simulink subsystem "StudentTemplate_MTMTAD006_M1(draft)"  (R2025a)
settings: Solver=VariableStepAuto  StartTime=0.0  StopTime=10.0  RelTol=1e-3
libraries: simulink x6, eeGeneralControl x3, slpidlib x1, cstblocks x1, dspstat3 x1
settings Model: Creator=JesseJabezArendse  LastModifiedBy=MTMTAD006

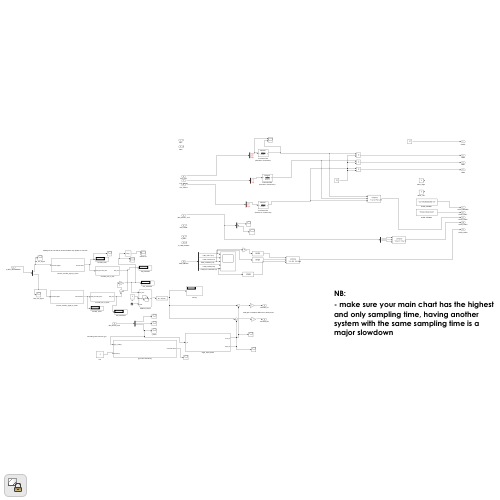
[thumbnail: Simulink's stored preview of the top-level diagram]
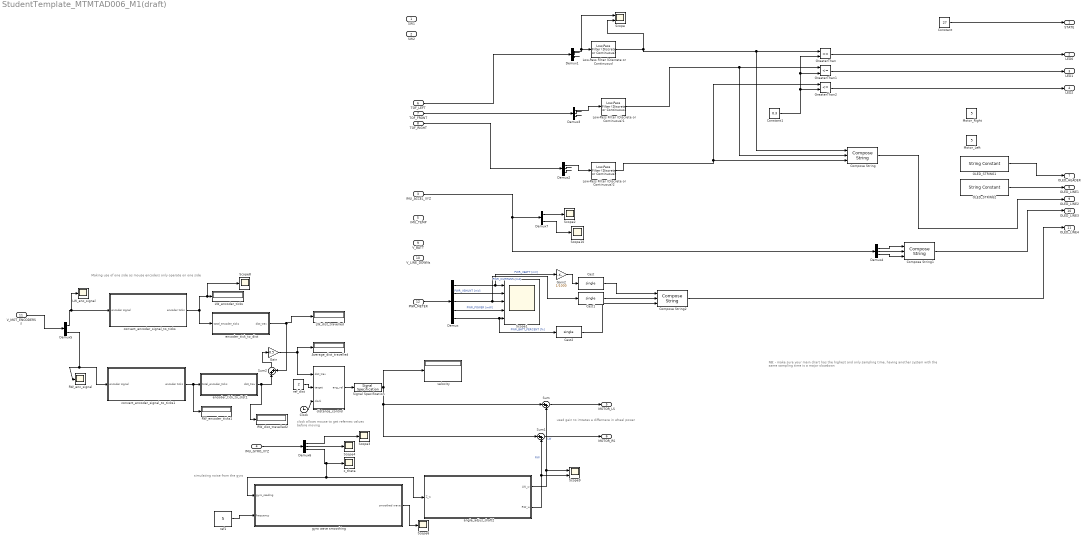
== system StudentTemplate_MTMTAD006_M1(draft) ==
  note: clock allows mouse to get refernec values
      | before moving
  note: used gain to imtates a differnece in wheel power
  note: simulating noise from the gyro
  note: Making use of one side as mouse encoders only operate on one side
  note: NB:
      |
      | - make sure your main chart has the highest and only sampling time, having another system with the same sampling time is a major slowdown
  SW1 : Inport
  SW2 : Inport  Port=2
  IMU_ACCEL_XYZ : Inport  Port=3
  IMU_GYRO_XYZ : Inport  Port=4
  IMU_TEMP : Inport  Port=5
  TOF_LEFT : Inport  Port=6
  TOF_FRONT : Inport  Port=7
  TOF_RIGHT : Inport  Port=8
  V_BATT : Inport  Port=9
  V_LINE_DOWNs : Inport  Port=10
  V_MOT_ENCODERSs : Inport  Port=11
  PWR_METER : Inport  Port=12
  Average_dist_travelled : Display
  Cast : DataTypeConversion  OutDataTypeStr=single  SaturateOnIntegerOverflow=off  RndMeth=Floor
  Cast1 : DataTypeConversion  OutDataTypeStr=single  SaturateOnIntegerOverflow=off  RndMeth=Floor
  Cast2 : DataTypeConversion  OutDataTypeStr=single  SaturateOnIntegerOverflow=off  RndMeth=Floor
  Clock : Clock
  Compose String : ComposeString  Format="\"L%1.2f F%1.2f R%1.2f\""
  Compose String1 : ComposeString  Format="\"X%2.1f  Y%2.1f  Z%2.1f\""
  Compose String2 : ComposeString  Format="\"%1.2fV  %3.0fmA  %2.0f%%\""
  Constant : Constant  Value=27
  Constant1 : Constant  Value=0.3  SampleTime=-1
  Demux : Demux  Outputs=5
  Demux{1..4,6..7} (6 alike) : Demux  Outputs=3
  Demux5 : Demux  Outputs=2
  Gain : Gain  Gain=0.5
  Gain2 : Gain  Gain=1/1000
  GreaterThan : RelationalOperator  Operator=<=  OutDataTypeStr=boolean  RndMeth=Simplest  InputSameDT=off
  GreaterThan1 : RelationalOperator  Operator=<=  OutDataTypeStr=boolean  RndMeth=Simplest  InputSameDT=off
  GreaterThan2 : RelationalOperator  Operator=<=  OutDataTypeStr=boolean  RndMeth=Simplest  InputSameDT=off
  LW_dist_travelled : Display
  LW_enc_signal : Scope
      settings: ActiveDisplayYMinimum=-1.5423087408726712  ActiveDisplayYMaximum=1.7466656009006407  DataLoggingVariableName=ScopeData3
  LW_encoder_ticks : Display
  Low-Pass Filter (Discrete or Continuous) : eeGeneralControl/Low-Pass Filter (Discrete or Continuous)  K=1  T=0.1  B=inf  A=-inf  init_option=Inherited from block input  x0=0  Ts=-1
  Low-Pass Filter (Discrete or Continuous)1 : eeGeneralControl/Low-Pass Filter (Discrete or Continuous)  K=1  T=0.1  B=inf  A=-inf  init_option=Inherited from block input  x0=0  Ts=-1
  Low-Pass Filter (Discrete or Continuous)2 : eeGeneralControl/Low-Pass Filter (Discrete or Continuous)  K=1  T=0.1  B=inf  A=-inf  init_option=Inherited from block input  x0=0  Ts=-1
  Motor_Left : Constant  Value=5
  Motor_Right : Constant  Value=5
  OLED_STRING1 : StringConstant  String="\"UCT MICROMOUSE '25\""
  OLED_STRING2 : StringConstant  String="\"Simulink Data Demo\""
  RW_dist_travelled2 : Display
  RW_enc_signal : Scope
      settings: ActiveDisplayYMinimum=-1.944570956862778  ActiveDisplayYMaximum=2.0482644886882531  DataLoggingVariableName=ScopeData4
  RW_encoder_ticks1 : Display
  Scope : Scope  NumInputPorts=2
      settings: ActiveDisplayYMinimum=0.22759  ActiveDisplayYMaximum=0.52326
  Scope1 : Scope  NumInputPorts=5
      settings: ActiveDisplayYMinimum=-437.5  ActiveDisplayYMaximum=3937.5  DataLoggingVariableName=ScopeData2
  Scope{2..4,6,8,10} (6 alike) : Scope
      Scope10 settings: ActiveDisplayYMinimum=-1.5661014992439717E+13  ActiveDisplayYMaximum=2.8937219425366357E+12  DataLoggingVariableName=ScopeData16
      Scope2 settings: ActiveDisplayYMinimum=-7.9001919672842393E+12  ActiveDisplayYMaximum=1.4712110348346104E+12
      Scope3 settings: ActiveDisplayYMinimum=-0.99701536683006531  ActiveDisplayYMaximum=1.0029846331699341  DataLoggingVariableName=ScopeData5
      Scope4 settings: ActiveDisplayYMinimum=-1.4593884470315912  ActiveDisplayYMaximum=1.2208028342184096  DataLoggingVariableName=ScopeData6
      Scope6 settings: ActiveDisplayYMinimum=-2.6130002287711669  ActiveDisplayYMaximum=3.775536484110495  DataLoggingVariableName=ScopeData11
      Scope8 settings: ActiveDisplayYMinimum=68.495784543089613  ActiveDisplayYMaximum=92.847652845801534  DataLoggingVariableName=ScopeData14
  Scope9 : Scope  NumInputPorts=2
      settings: ActiveDisplayYMinimum=-3.4090236125299427  ActiveDisplayYMaximum=2.7340238993056811  DataLoggingVariableName=ScopeData17
  Signal Specification : SignalSpecification  Dimensions=1  SampleTime=0.05
  Sum : Sum  Inputs=|++
  Sum1 : Sum  Inputs=|++
  Sum2 : Sum  Inputs=|++
  angle_adjus_draft2 : Subsystem
  convert_encoder_signal_to_ticks : Subsystem
  convert_encoder_signal_to_ticks1 : Subsystem
  distance_control : Stateflow chart  TreatAsAtomicUnit=on
  encoder_tick_to_dist : Subsystem
  encoder_tick_to_dist1 : Subsystem
  "gyro wave smoothing " : Subsystem
  ref1 : Constant  Value=5
  ref_dist : Constant  Value=2
  velocity : Display
  z_theta : Scope
      settings: ActiveDisplayYMinimum=-0.11007907923009226  ActiveDisplayYMaximum=0.2597891347301477  DataLoggingVariableName=ScopeData7
  STATE : Outport
  LED0 : Outport  Port=2
  LED1 : Outport  Port=3
  LED2 : Outport  Port=4
  MOTOR_LS : Outport  Port=5
  MOTOR_RS : Outport  Port=6
  OLED_HEADER : Outport  Port=7
  OLED_LINE1 : Outport  Port=8
  OLED_LINE2 : Outport  Port=9
  OLED_LINE3 : Outport  Port=10
  OLED_LINE4 : Outport  Port=11
  wires:
  TOF_FRONT/1 -> Demux3/1
  OLED_STRING2/1 -> OLED_LINE1/1
  Demux2/1 -> Low-Pass Filter (Discrete or Continuous)2/1
  Demux2/3 -> ?
  Demux2/2 -> ?
  ? -> ?
  Compose String1/1 -> OLED_LINE3/1
  Low-Pass Filter (Discrete or Continuous)1/1 -> Compose String/2, GreaterThan1/1
  GreaterThan1/1 -> LED1/1
  Demux3/3 -> ?
  TOF_RIGHT/1 -> Demux2/1
  ? -> ?
  Demux3/2 -> ?
  Demux1/2 -> ?
  Demux3/1 -> Low-Pass Filter (Discrete or Continuous)1/1
  OLED_STRING1/1 -> OLED_HEADER/1
  Demux1/1 -> Scope/1, Low-Pass Filter (Discrete or Continuous)/1
  Compose String/1 -> OLED_LINE2/1
  Constant1/1 -> GreaterThan2/2, GreaterThan1/2, GreaterThan/2
  ? -> ?
  GreaterThan2/1 -> LED2/1
  TOF_LEFT/1 -> Demux1/1
  GreaterThan/1 -> LED0/1
  Demux1/3 -> ?
  PWR_METER/1 -> Demux/1
  Demux/1 -> Scope1/1, Gain2/1  "PWR_VBATT [mV]"
  Demux/2 -> Scope1/2  "PWR_VSHUNT [mV]"
  Demux/3 -> Scope1/3, Cast1/1  "PWR_CURRENT [mA]"
  Demux/4 -> Scope1/4  "PWR_POWER [mW]"
  Demux/5 -> Scope1/5, Cast2/1  "PWR_BATT_PERCENT [%]"
  IMU_ACCEL_XYZ/1 -> Demux7/1, Demux4/1
  Demux4/1 -> Compose String1/1
  Demux4/2 -> Compose String1/2
  Demux4/3 -> Compose String1/3
  Compose String2/1 -> OLED_LINE4/1
  Gain2/1 -> Cast/1
  Cast/1 -> Compose String2/1
  Cast1/1 -> Compose String2/2
  Cast2/1 -> Compose String2/3
  Low-Pass Filter (Discrete or Continuous)2/1 -> Compose String/3, GreaterThan2/1
  Low-Pass Filter (Discrete or Continuous)/1 -> Scope/2, Compose String/1, GreaterThan/1
  Constant/1 -> STATE/1
  V_MOT_ENCODERSs/1 -> Demux5/1
  Demux5/1 -> LW_enc_signal/1, convert_encoder_signal_to_ticks/1(encoder signal)
  Demux5/2 -> convert_encoder_signal_to_ticks1/1(encoder signal), RW_enc_signal/1
  convert_encoder_signal_to_ticks/1(encoder ticks) -> LW_encoder_ticks/1, Scope8/1, encoder_tick_to_dist/1(total_encoder_ticks)
  encoder_tick_to_dist/1(dist_trav) -> Sum2/2, LW_dist_travelled/1
  ref_dist/1 -> distance_control/2(target)
  distance_control/1(ang_vel) -> Signal Specification/1
  IMU_GYRO_XYZ/1 -> Demux6/1
  Signal Specification/1 -> Sum/1, Sum1/1, velocity/1
  Demux6/1 -> Scope3/1
  Demux6/2 -> Scope4/1
  Demux6/3 -> z_theta/1, "gyro wave smoothing "/1(gyro_reading), angle_adjus_draft2/1(Z_w)
  ref1/1 -> "gyro wave smoothing "/2(frequency)
  "gyro wave smoothing "/1(smoothed wave) -> Scope6/1
  convert_encoder_signal_to_ticks1/1(encoder ticks) -> encoder_tick_to_dist1/1(total_encoder_ticks), RW_encoder_ticks1/1
  encoder_tick_to_dist1/1(dist_trav) -> Sum2/1, RW_dist_travelled2/1
  Sum2/1 -> Gain/1
  Sum/1 -> MOTOR_LS/1
  Clock/1 -> distance_control/3(clock)
  Sum1/1 -> MOTOR_RS/1
  Gain/1 -> Average_dist_travelled/1, distance_control/1(dist_trav)
  Demux7/1 -> Scope2/1
  Demux7/3 -> Scope10/1
  angle_adjus_draft2/1(LW_w) -> Scope9/1, Sum/2  "LW"
  angle_adjus_draft2/2(RW_w) -> Scope9/2, Sum1/2  "RW"

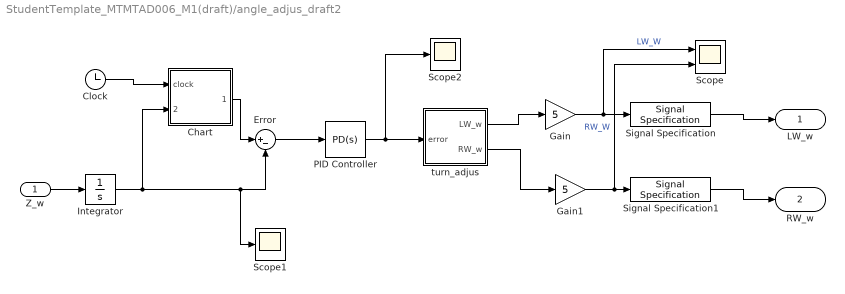
== system StudentTemplate_MTMTAD006_M1(draft)/angle_adjus_draft2 ==
  Z_w : Inport
  Chart : Stateflow chart  TreatAsAtomicUnit=on
  Clock : Clock
  Error : Sum  Inputs=|+-
  Gain : Gain  Gain=5
  Gain1 : Gain  Gain=5
  Integrator : Integrator
  PID Controller : slpidlib/PID Controller  Controller=PD  Form=Parallel  TimeDomain=Continuous-time  UseExternalTs=off  SampleTime=-1  IntegratorMethod=Forward Euler  FilterMethod=Forward Euler  ControllerParametersSource=internal  P=50  I=1  UseKiTs=off  D=1  UseExternalDerivativeSource=off  N=100  UseFilter=on  TunerSelectOption=Transfer Function Based (PID Tuner App)  InitialConditionSource=internal  InitialConditionForIntegrator=0  InitialConditionForFilter=0  DifferentiatorICPrevScaledInput=0  ExternalReset=none  TrackingMode=off  Kt=1  LimitOutput=off  SatLimitsSource=internal  UpperSaturationLimit=inf  LowerSaturationLimit=-inf  LinearizeAsGain=on  AntiWindupMode=none  Kb=1  LimitIntegrator=off  UpperIntegratorSaturationLimit=inf  LowerIntegratorSaturationLimit=-inf  POutMin=[]  POutMax=[]  IOutMin=[]  IOutMax=[]  DOutMin=[]  DOutMax=[]  NOutMin=[]  NOutMax=[]  SumOutMin=[]  SumOutMax=[]  SaturationOutMin=[]  SaturationOutMax=[]  PParamMin=[]  PParamMax=[]  IParamMin=[]  IParamMax=[]  DParamMin=[]  DParamMax=[]  NParamMin=[]  NParamMax=[]  KbParamMin=[]  KbParamMax=[]  KtParamMin=[]  KtParamMax=[]  KbOutMin=[]  KbOutMax=[]  KtOutMin=[]  KtOutMax=[]  IntegratorOutMin=[]  IntegratorOutMax=[]  FilterOutMin=[]  FilterOutMax=[]  SumI1OutMin=[]  SumI1OutMax=[]  SumI2OutMin=[]  SumI2OutMax=[]  SumI3OutMin=[]  SumI3OutMax=[]  SumI4OutMin=[]  SumI4OutMax=[]  SumDOutMin=[]  SumDOutMax=[]  DifferentiatorOutMin=[]  DifferentiatorOutMax=[]  FilterDiffOutCoefMin=[]  FilterDiffOutCoefMax=[]  ReciprocalOutMin=[]  ReciprocalOutMax=[]  SumDenOutMin=[]  SumDenOutMax=[]  SumNumOutMin=[]  SumNumOutMax=[]  DivideOutMin=[]  DivideOutMax=[]  UdiffTsProdOutMin=[]  UdiffTsProdOutMax=[]  NTsProdOutMin=[]  NTsProdOutMax=[]  UintegralTsProdOutMin=[]  UintegralTsProdOutMax=[]  UngainTsProdOutMin=[]  UngainTsProdOutMax=[]  ClampingZeroOutDataTypeStr=Inherit: Inherit via back propagation  ClampingZeroOutMin=[]  ClampingZeroOutMax=[]  FilterDenConstantOutDataTypeStr=Inherit: Inherit via back propagation  FilterDenConstantOutMin=[]  FilterDenConstantOutMax=[]  PCopyOutDataTypeStr=Inherit: Inherit via back propagation  PCopyOutMin=[]  PCopyOutMax=[]  NCopyOutDataTypeStr=Inherit: Inherit via back propagation  NCopyOutMin=[]  NCopyOutMax=[]  IntegratorContinuousStateAttributes=''  IntegratorStateMustResolveToSignalObject=off  IntegratorRTWStateStorageClass=Auto  FilterContinuousStateAttributes=''  FilterStateMustResolveToSignalObject=off  FilterRTWStateStorageClass=Auto  ParallelPVariant=InternalParameters  IdealPVariant=Disabled  IVariant=Disabled  DVariant=InternalParameters  IntegratorVariant=Disabled  SatVariant=Disabled  AWVariant=Disabled  PCopyVariant=Disabled  TRVariant=Disabled  FdbkBlocksVariant=Forward  IdealPFdbkVariant=Disabled  SatFdbkVariant=Disabled  DerivativeFilterVariant=ContFilter  NVariant=InternalParameters  NCopyVariant=Disabled  FilterICVariant=InternalICsFilter  IntegratorICVariant=Disabled  ExternalResetVariant=Disabled  TRSumVariant=Passthrough  SumFdbkVariant=Disabled  SumVariant=Sum_PD  TsampFilterVariant=InternalTs  TsampNgainVariant=Passthrough  TsampIntegralVariant=Disabled_SignalSpec  ExternalSaturationOutDataTypeStr=Inherit: Same as second input  DerivativeSourceVariant=ErrorSignal  PreIntVariant=InternalPreInt
  Scope : Scope  NumInputPorts=2
      settings: ActiveDisplayYMinimum=-440.40684872460486  ActiveDisplayYMaximum=398.93122569343797  DataLoggingVariableName=ScopeData8
  Scope1 : Scope
      settings: ActiveDisplayYMinimum=-2.1976138852237335  ActiveDisplayYMaximum=0.12970641062525379  DataLoggingVariableName=ScopeData12
  Scope2 : Scope
      settings: ActiveDisplayYMinimum=-4.4488284675734473  ActiveDisplayYMaximum=3.9249085751009725  DataLoggingVariableName=ScopeData10
  Signal Specification : SignalSpecification  Dimensions=1
  Signal Specification1 : SignalSpecification  Dimensions=1
  turn_adjus : Stateflow chart  TreatAsAtomicUnit=on
  LW_w : Outport
  RW_w : Outport  Port=2
  wires:
  Clock/1 -> Chart/1(clock)
  Gain1/1 -> Signal Specification1/1, Scope/2  "RW_W"
  Gain/1 -> Signal Specification/1, Scope/1  "LW_W"
  Chart/1(offset) -> Error/1
  Z_w/1 -> Integrator/1
  Signal Specification1/1 -> RW_w/1
  Signal Specification/1 -> LW_w/1
  turn_adjus/2(RW_w) -> Gain1/1
  turn_adjus/1(LW_w) -> Gain/1
  PID Controller/1 -> turn_adjus/1(error), Scope2/1
  Error/1 -> PID Controller/1
  Integrator/1 -> Error/2, Scope1/1, Chart/2(Z_theta)

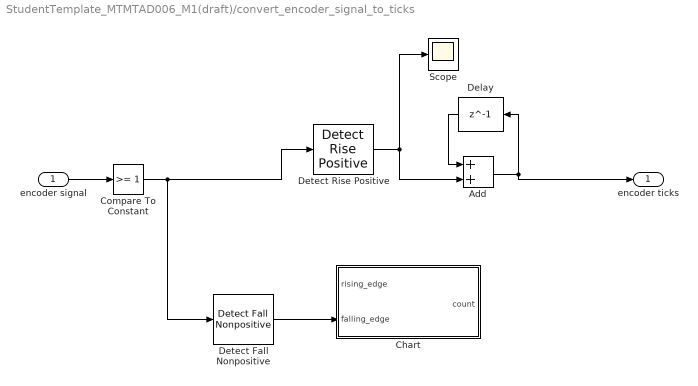
== system StudentTemplate_MTMTAD006_M1(draft)/convert_encoder_signal_to_ticks ==
  encoder signal : Inport
  Add : Sum
  Chart : Stateflow chart  TreatAsAtomicUnit=on
  Compare To Constant : simulink/Logic and Bit Operations/Compare To Constant  relop=>=  const=1  OutDataTypeStr=boolean
  Delay : Delay  DelayLength=1  InitialCondition=0
  Detect Fall Nonpositive : simulink/Logic and Bit Operations/Detect Fall Nonpositive  vinit=0  OutDataTypeStr=boolean
  Detect Rise Positive : simulink/Logic and Bit Operations/Detect Rise Positive  vinit=0  OutDataTypeStr=uint8
  Scope : Scope
      settings: ActiveDisplayYMinimum=-0.30381603839463822  ActiveDisplayYMaximum=1.4550594899256748  DataLoggingVariableName=ScopeData9
  encoder ticks : Outport
  wires:
  Detect Fall Nonpositive/1 -> Chart/2(falling_edge)
  Delay/1 -> Add/1
  encoder signal/1 -> Compare To Constant/1
  Detect Rise Positive/1 -> Scope/1, Add/2
  Compare To Constant/1 -> Detect Rise Positive/1, Detect Fall Nonpositive/1
  Add/1 -> Delay/1, encoder ticks/1

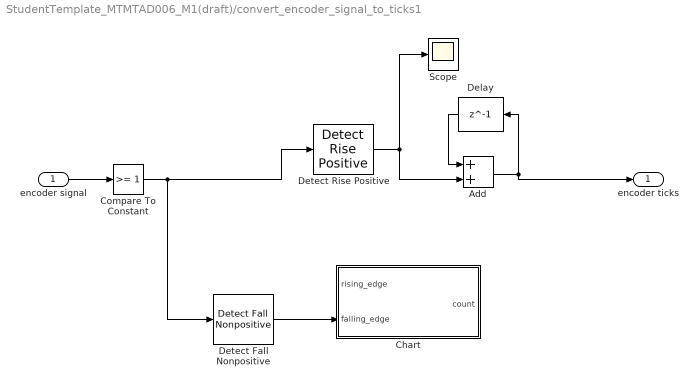
== system StudentTemplate_MTMTAD006_M1(draft)/convert_encoder_signal_to_ticks1 ==
  encoder signal : Inport
  Add : Sum
  Chart : Stateflow chart  TreatAsAtomicUnit=on
  Compare To Constant : simulink/Logic and Bit Operations/Compare To Constant  relop=>=  const=1  OutDataTypeStr=boolean
  Delay : Delay  DelayLength=1  InitialCondition=0
  Detect Fall Nonpositive : simulink/Logic and Bit Operations/Detect Fall Nonpositive  vinit=0  OutDataTypeStr=boolean
  Detect Rise Positive : simulink/Logic and Bit Operations/Detect Rise Positive  vinit=0  OutDataTypeStr=uint8
  Scope : Scope
      settings: ActiveDisplayYMinimum=-0.30381603839463822  ActiveDisplayYMaximum=1.4550594899256748  DataLoggingVariableName=ScopeData9
  encoder ticks : Outport
  wires:
  Detect Fall Nonpositive/1 -> Chart/2(falling_edge)
  Delay/1 -> Add/1
  encoder signal/1 -> Compare To Constant/1
  Detect Rise Positive/1 -> Scope/1, Add/2
  Compare To Constant/1 -> Detect Rise Positive/1, Detect Fall Nonpositive/1
  Add/1 -> Delay/1, encoder ticks/1

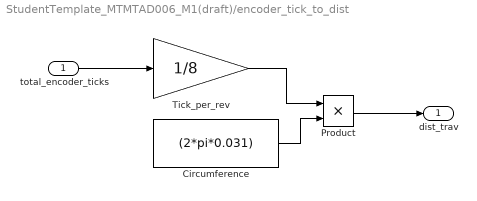
== system StudentTemplate_MTMTAD006_M1(draft)/encoder_tick_to_dist ==
  total_encoder_ticks : Inport
  Circumference : Constant  Value=(2*pi*0.031)
  Product : Product
  Tick_per_rev : Gain  Gain=1/8
  dist_trav : Outport
  wires:
  total_encoder_ticks/1 -> Tick_per_rev/1
  Circumference/1 -> Product/2
  Tick_per_rev/1 -> Product/1
  Product/1 -> dist_trav/1

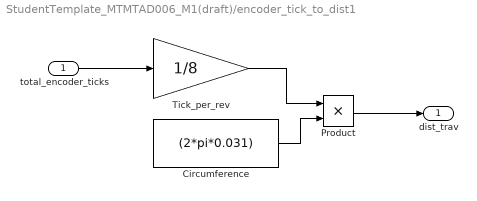
== system StudentTemplate_MTMTAD006_M1(draft)/encoder_tick_to_dist1 ==
  total_encoder_ticks : Inport
  Circumference : Constant  Value=(2*pi*0.031)
  Product : Product
  Tick_per_rev : Gain  Gain=1/8
  dist_trav : Outport
  wires:
  total_encoder_ticks/1 -> Tick_per_rev/1
  Circumference/1 -> Product/2
  Tick_per_rev/1 -> Product/1
  Product/1 -> dist_trav/1

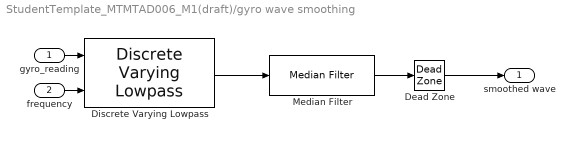
== system StudentTemplate_MTMTAD006_M1(draft)/gyro wave smoothing  ==
  gyro_reading : Inport
  frequency : Inport  Port=2
  Dead Zone : DeadZone
  Discrete Varying Lowpass : cstblocks/Linear Parameter Varying/Discrete Varying Lowpass  N=4  w0=0  Ts=0.01
  Median Filter : dspstat3/Median Filter  WindowLength=5  SimulateUsing=Interpreted execution
      settings: LibrarySourceBlock=|
      | dspfdesign/Median
      | Filter
  smoothed wave : Outport
  wires:
  gyro_reading/1 -> Discrete Varying Lowpass/1
  Dead Zone/1 -> smoothed wave/1
  frequency/1 -> Discrete Varying Lowpass/2
  Discrete Varying Lowpass/1 -> Median Filter/1
  Median Filter/1 -> Dead Zone/1

== stateflow chart StudentTemplate_MTMTAD006_M1(draft)/angle_adjus_draft2/turn_adjus ==
  state deafult
    during:
    LW_w = 0;
    RW_w = 0;
  state turnLeft
    during:
    LW_w=-error;
    RW_w = error;
  state turnRight
    during:
    RW_w = error;
    LW_w = -error;
  (default) -> deafult
  deafult -> turnLeft [order 2] : [error>0 ]
  deafult -> turnRight [order 1] : [error<0 ]
  data: error input; LW_w output; RW_w output; err local

== stateflow chart StudentTemplate_MTMTAD006_M1(draft)/angle_adjus_draft2/Chart ==
  state Start
    during:
    offset= 0;
  state Set_Offset
    during:
    offset = Z_theta;
  (default) -> Start
  Start -> Set_Offset : [clock <0.1]
  Set_Offset -> Set_Offset : [clock > 0.1]
  data: clock input; offset output; Z_theta input

== stateflow chart StudentTemplate_MTMTAD006_M1(draft)/distance_control ==
  state start
    ang_vel = 0;
  state Run
    during:
    ang_vel = 50;
  state Stop
    during:
    ang_vel =0;
  (default) -> start
  Run -> Stop : [dist_trav>= target ]
  start -> Run : [clock > 5]
  data: dist_trav input; target input; ang_vel output; clock input

== stateflow chart StudentTemplate_MTMTAD006_M1(draft)/convert_encoder_signal_to_ticks/Chart ==
  state default
    during:
    count =0;
  state encoder_pulse_start
    during:
  state encoder_pulse_end
    during:
    count = 1;
  (default) -> default
  default -> encoder_pulse_start : [rising_edge == 1]
  encoder_pulse_start -> encoder_pulse_end : [falling_edge == 1]
  data: rising_edge input; count output; falling_edge input

== stateflow chart StudentTemplate_MTMTAD006_M1(draft)/convert_encoder_signal_to_ticks1/Chart ==
  state default
    during:
    count =0;
  state encoder_pulse_start
    during:
  state encoder_pulse_end
    during:
    count = 1;
  (default) -> default
  default -> encoder_pulse_start : [rising_edge == 1]
  encoder_pulse_start -> encoder_pulse_end : [falling_edge == 1]
  data: rising_edge input; count output; falling_edge input
